simulink model "mat_mult_test"  (Simulink 4.00)
settings: Solver=ode45  StartTime=0.0  StopTime=10.0  RelTol=1e-3
settings Model: Creator=mcar  LastModifiedBy=mcar  BlockReductionOpt=off

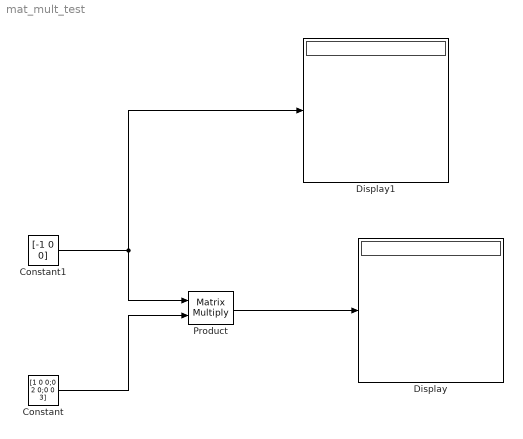
== system mat_mult_test ==
  Constant : Constant  Value=[1 0 0;0 2 0;0 0 3]
  Constant1 : Constant  Value=[-1 0 0]  VectorParams1D=off
  Display : Display
      settings: Format=short
  Display1 : Display
      settings: Format=short
  Product : Product  Inputs=2  Multiplication=Matrix(*)  SaturateOnIntegerOverflow=on
  wires:
  Constant1/1 -> Display1/1, Product/1
  Constant/1 -> Product/2
  Product/1 -> Display/1
